simulink model "network_model"  (R2022b)
settings: Solver=ode23t  StartTime=0.0  StopTime=50  FixedStep=1e-3  RelTol=1e-3
values from neighbouring files (symbols this model uses):
  a = 0.9    [network_control.m]
  B = 8    [network_control.m]
  C = 6    [network_control.m]
  k1 = 0.4    [network_control.m]
  k2 = 0.8    [network_control.m]
  k3 = 0.1    [network_control.m]
  q_i_1 = [-2 2 0]'    [network_control.m]
  q_i_2 = [-4 4 0]'    [network_control.m]
  taup = 0    [network_control.m]
  Ts = 0.01    [network_control.m]
libraries: robotmobilelib x2
settings Model: Creator=danie  LastModifiedBy=gaetano
settings OptimizationCC: ReuseModelBlockBuffer=on

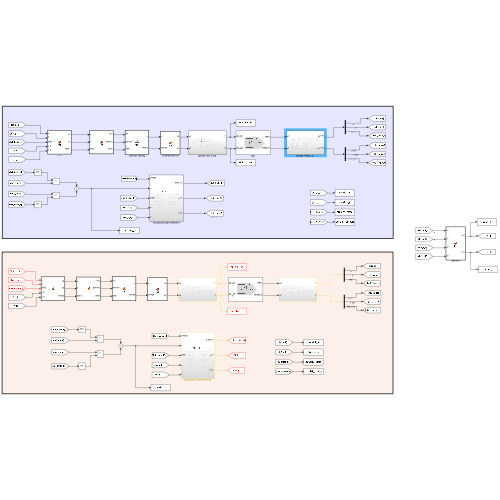
[thumbnail: Simulink's stored preview of the top-level diagram]
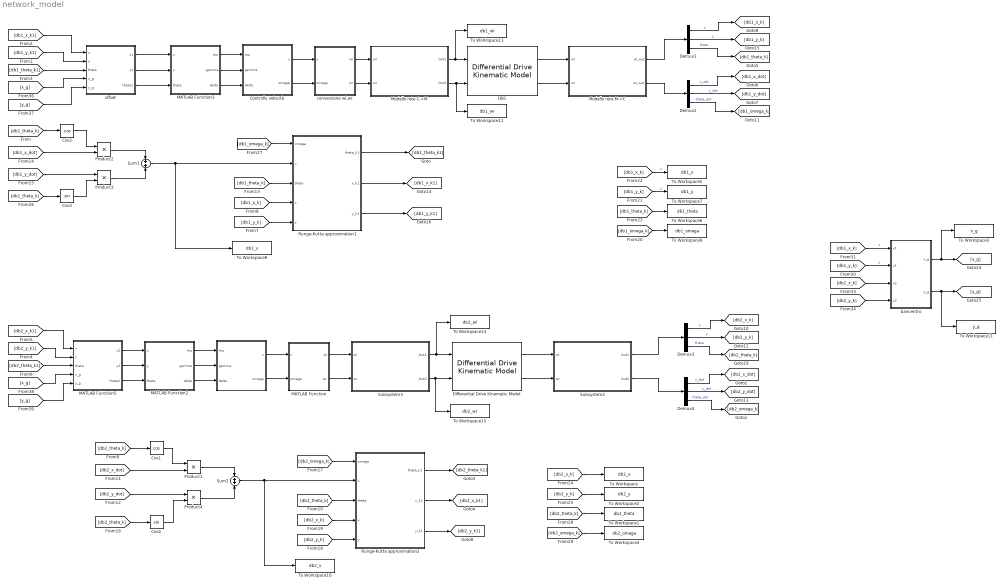
== system network_model ==
  " " : MATLAB Function  TreatAsAtomicUnit=on
  " Controllo velocità" : MATLAB Function  TreatAsAtomicUnit=on
  Cos1 : Trigonometry  Operator=cos
  Cos2 : Trigonometry  Operator=cos
  Cos3 : Trigonometry
  Cos4 : Trigonometry
  DB1 : robotmobilelib/Differential Drive Kinematic Model  VehicleInputs=Wheel Speeds  WheelRadius=0.0318  WheelSpeedRange=[-inf inf]  TrackWidth=0.1232  InitialState=q_i_1  SimulateUsing=Code generation
  Demux{1..4} (4 alike) : Demux  Outputs=3
  Differential Drive Kinematic Model : robotmobilelib/Differential Drive Kinematic Model  VehicleInputs=Wheel Speeds  WheelRadius=0.0318  WheelSpeedRange=[-inf inf]  TrackWidth=0.1232  InitialState=q_i_2  SimulateUsing=Interpreted execution
  MATLAB Function : MATLAB Function  TreatAsAtomicUnit=on
  MATLAB Function2 : MATLAB Function  TreatAsAtomicUnit=on
  MATLAB Function3 : MATLAB Function  TreatAsAtomicUnit=on
  MATLAB Function5 : MATLAB Function  TreatAsAtomicUnit=on
  Modello rete C->M : Subsystem
  Modello rete M->C : Subsystem
  Product{1..4} (4 alike) : Product
  Runge-Kutta approximation1 : Subsystem
  Runge-Kutta approximation2 : Subsystem
  Subsystem2 : Subsystem
  Subsystem3 : Subsystem
  Sum1 : Sum  Inputs=+|+
  Sum2 : Sum  Inputs=+|+
  To Workspace : ToWorkspace  VariableName=db2_x  SaveFormat=Timeseries  SampleTime=-1
  To Workspace1 : ToWorkspace  VariableName=db2_theta  SaveFormat=Timeseries  SampleTime=-1
  To Workspace10 : ToWorkspace  VariableName=db2_v  SaveFormat=Timeseries  SampleTime=-1
  To Workspace11 : ToWorkspace  VariableName=y_g  SaveFormat=Timeseries  SampleTime=-1
  To Workspace12 : ToWorkspace  VariableName=db1_wr  SaveFormat=Timeseries  SampleTime=-1
  To Workspace13 : ToWorkspace  VariableName=db1_wl  SaveFormat=Timeseries  SampleTime=-1
  To Workspace14 : ToWorkspace  VariableName=db2_wl  SaveFormat=Timeseries  SampleTime=-1
  To Workspace15 : ToWorkspace  VariableName=db2_wr  SaveFormat=Timeseries  SampleTime=-1
  To Workspace2 : ToWorkspace  VariableName=db2_y  SaveFormat=Timeseries  SampleTime=-1
  To Workspace3 : ToWorkspace  VariableName=x_g  SaveFormat=Timeseries  SampleTime=-1
  To Workspace4 : ToWorkspace  VariableName=db2_omega  SaveFormat=Timeseries  SampleTime=-1
  To Workspace5 : ToWorkspace  VariableName=db1_x  SaveFormat=Timeseries  SampleTime=-1
  To Workspace6 : ToWorkspace  VariableName=db1_theta  SaveFormat=Timeseries  SampleTime=-1
  To Workspace7 : ToWorkspace  VariableName=db1_y  SaveFormat=Timeseries  SampleTime=-1
  To Workspace8 : ToWorkspace  VariableName=db1_v  SaveFormat=Timeseries  SampleTime=-1
  To Workspace9 : ToWorkspace  VariableName=db1_omega  SaveFormat=Timeseries  SampleTime=-1
  baricentro : MATLAB Function  TreatAsAtomicUnit=on
  conversione wl,wr : MATLAB Function  TreatAsAtomicUnit=on
  offset : MATLAB Function  TreatAsAtomicUnit=on
  wires:
  MATLAB Function3/3(delta) -> " Controllo velocità"/3(delta)
  [db1_theta_k] -> To Workspace6/1
  [db2_y_k] -> Runge-Kutta approximation2/5(y)
  Runge-Kutta approximation2/2(x_k1) -> [db2_x_k1]
  " "/2(omega) -> MATLAB Function/2(omega)
  [db1_y_k] -> Runge-Kutta approximation1/5(y)
  Runge-Kutta approximation2/3(y_k1) -> [db2_y_k1]
  Demux2/1 -> [db1_x_dot]  "x_dot"
  [db1_omega_k] -> Runge-Kutta approximation1/1(omega)
  [db1_theta_k] -> Cos2/1
  Demux1/3 -> [db1_theta_k]  "theta"
  [db1_theta_k] -> Cos3/1
  Product1/1 -> Sum2/1
  Cos1/1 -> Product1/1
  Cos3/1 -> Product3/2
  [db2_theta_k] -> Runge-Kutta approximation2/3(theta)
  Product4/1 -> Sum2/2
  Cos4/1 -> Product4/2
  " Controllo velocità"/1(v) -> conversione wl,wr/1(v)
  Demux1/2 -> [db1_y_k]  "y"
  Demux2/3 -> [db1_omega_k]  "theta_dot"
  Cos2/1 -> Product2/1
  offset/2(y1) -> MATLAB Function3/2(y)
  Demux1/1 -> [db1_x_k]  "x"
  [db1_x_dot] -> Product2/2
  [db1_x_k] -> Runge-Kutta approximation1/4(x)
  Runge-Kutta approximation1/1(theta_k1) -> [db1_theta_k1]
  MATLAB Function3/1(rho) -> " Controllo velocità"/1(rho)
  MATLAB Function2/2(gamma) -> " "/2(gamma)
  " "/1(v) -> MATLAB Function/1(v)
  Demux4/1 -> [db2_x_dot]  "x_dot"
  Product3/1 -> Sum1/2
  [db2_y_k] -> To Workspace2/1
  Sum2/1 -> To Workspace10/1, Runge-Kutta approximation2/2(v)
  [db1_theta_k] -> Runge-Kutta approximation1/3(theta)
  Product2/1 -> Sum1/1
  Demux3/1 -> [db2_x_k]  "x"
  [db2_theta_k] -> Cos4/1
  offset/3(theta1) -> MATLAB Function3/3(theta)
  [db1_y_k] -> baricentro/2(y1)  "y"
  [db1_x_k] -> baricentro/1(x1)  "x"
  MATLAB Function2/1(rho) -> " "/1(rho)
  Sum1/1 -> To Workspace8/1, Runge-Kutta approximation1/2(v)
  [db2_x_k] -> baricentro/3(x2)
  Demux4/3 -> [db2_omega_k]  "theta_dot"
  [db2_omega_k] -> To Workspace4/1
  " Controllo velocità"/2(omega) -> conversione wl,wr/2(omega)
  [db1_y_k1] -> offset/2(y)
  [db2_omega_k] -> Runge-Kutta approximation2/1(omega)
  Demux3/3 -> [db2_theta_k]  "theta"
  [db2_theta_k1] -> MATLAB Function5/3(theta)
  [db2_y_k1] -> MATLAB Function5/2(y)
  MATLAB Function5/1(x2) -> MATLAB Function2/1(x)
  MATLAB Function3/2(gamma) -> " Controllo velocità"/2(gamma)
  [db1_x_k] -> To Workspace5/1  "x"
  [y_g] -> offset/5(y_g)
  [db2_x_k] -> To Workspace/1
  [db1_x_k1] -> offset/1(x)
  Runge-Kutta approximation1/3(y_k1) -> [db1_y_k1]
  [x_g] -> offset/4(x_g)
  [db2_x_k1] -> MATLAB Function5/1(x)
  [db1_y_dot] -> Product3/1
  MATLAB Function5/2(y2) -> MATLAB Function2/2(y)
  [y_g] -> MATLAB Function5/5(y_g)
  [db2_theta_k] -> To Workspace1/1
  [db1_y_k] -> To Workspace7/1  "y"
  [x_g] -> MATLAB Function5/4(x_g)
  [db1_theta_k1] -> offset/3(theta)
  offset/1(x1) -> MATLAB Function3/1(x)
  baricentro/2(y_g) -> [y_g], To Workspace11/1
  [db2_x_k] -> Runge-Kutta approximation2/4(x)
  Demux3/2 -> [db2_y_k]  "y"
  [db2_y_dot] -> Product4/1
  [db2_theta_k] -> Cos1/1
  Demux4/2 -> [db2_y_dot]  "y_dot"
  [db1_omega_k] -> To Workspace9/1
  Runge-Kutta approximation1/2(x_k1) -> [db1_x_k1]
  Demux2/2 -> [db1_y_dot]  "y_dot"
  [db2_x_dot] -> Product1/2
  MATLAB Function2/3(delta) -> " "/3(delta)
  Runge-Kutta approximation2/1(theta_k1) -> [db2_theta_k1]
  baricentro/1(x_g) -> [x_g], To Workspace3/1
  MATLAB Function5/3(theta2) -> MATLAB Function2/3(theta)
  [db2_y_k] -> baricentro/4(y2)
  conversione wl,wr/1(wl) -> Modello rete C->M/1(wl)
  conversione wl,wr/2(wr) -> Modello rete C->M/2(wr)
  Modello rete C->M/1(Out1) -> To Workspace13/1, DB1/1
  Modello rete C->M/2(Out2) -> To Workspace12/1, DB1/2
  Modello rete M->C/1(wl_out) -> Demux1/1
  Modello rete M->C/2(wr_out) -> Demux2/1
  DB1/1 -> Modello rete M->C/1(wl)
  DB1/2 -> Modello rete M->C/2(wr)
  Subsystem2/1(Out1) -> Demux3/1
  Subsystem2/2(Out2) -> Demux4/1
  Differential Drive Kinematic Model/2 -> Subsystem2/2(wr)
  Differential Drive Kinematic Model/1 -> Subsystem2/1(wl)
  MATLAB Function/1(wl) -> Subsystem3/1(wl)
  MATLAB Function/2(wr) -> Subsystem3/2(wr)
  Subsystem3/2(Out2) -> To Workspace15/1, Differential Drive Kinematic Model/2
  Subsystem3/1(Out1) -> To Workspace14/1, Differential Drive Kinematic Model/1

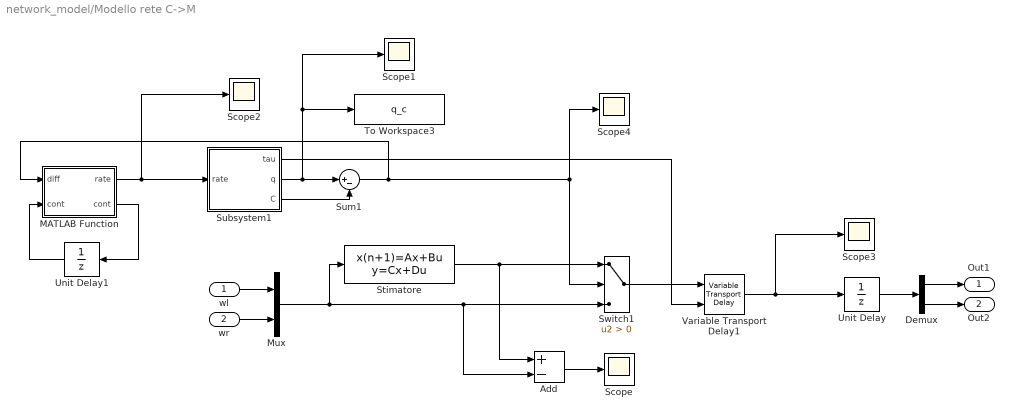
== system network_model/Modello rete C->M ==
  wl : Inport
  wr : Inport  Port=2
  Add : Sum  Inputs=+-
  Demux : Demux  Outputs=2
  MATLAB Function : MATLAB Function  TreatAsAtomicUnit=on
  Mux : Mux  Inputs=2
  Scope{,1..4} (5 alike) : Scope
  Stimatore : DiscreteStateSpace  A=(1-a)*eye(2)  B=a*eye(2)  C=eye(2)  D=zeros(2,2)  SampleTime=-1
  Subsystem1 : Subsystem
  Sum1 : Sum  Inputs=|+-
  Switch1 : Switch  Criteria=u2 > Threshold  SaturateOnIntegerOverflow=off  InputSameDT=off
  To Workspace3 : ToWorkspace  VariableName=q_c  SaveFormat=Timeseries  SampleTime=-1
  Unit Delay : UnitDelay  SampleTime=0.01  HasFrameUpgradeWarning=on
  Unit Delay1 : UnitDelay  SampleTime=-1  HasFrameUpgradeWarning=on
  Variable Transport Delay1 : VariableTransportDelay  MaximumDelay=10  MaximumPoints=2048  ZeroDelay=on
  Out1 : Outport
  Out2 : Outport  Port=2
  wires:
  Switch1/1 -> Variable Transport Delay1/1
  Subsystem1/3(C) -> Sum1/2
  Subsystem1/1(tau) -> Variable Transport Delay1/2
  Subsystem1/2(q) -> To Workspace3/1, Scope1/1, Sum1/1
  Sum1/1 -> MATLAB Function/1(diff), Scope4/1, Switch1/2
  wl/1 -> Mux/1
  wr/1 -> Mux/2
  Mux/1 -> Stimatore/1, Add/2, Switch1/3
  Variable Transport Delay1/1 -> Scope3/1, Unit Delay/1
  Demux/1 -> Out1/1
  Demux/2 -> Out2/1
  Unit Delay/1 -> Demux/1
  Stimatore/1 -> Switch1/1, Add/1
  Add/1 -> Scope/1
  MATLAB Function/1(rate) -> Scope2/1, Subsystem1/1(rate)
  MATLAB Function/2(cont) -> Unit Delay1/1
  Unit Delay1/1 -> MATLAB Function/2("cont ")

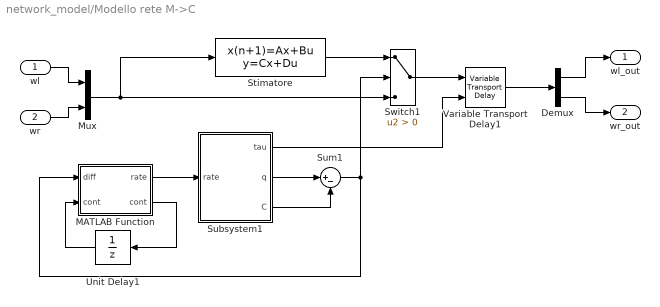
== system network_model/Modello rete M->C ==
  wl : Inport
  wr : Inport  Port=2
  Demux : Demux  Outputs=2
  MATLAB Function : MATLAB Function  TreatAsAtomicUnit=on
  Mux : Mux  Inputs=2
  Stimatore : DiscreteStateSpace  A=(1-a)*eye(6)  B=a*eye(6)  C=eye(6)  D=zeros(6,6)  SampleTime=-1
  Subsystem1 : Subsystem
  Sum1 : Sum  Inputs=|+-
  Switch1 : Switch  Criteria=u2 > Threshold  SaturateOnIntegerOverflow=off  InputSameDT=off
  Unit Delay1 : UnitDelay  SampleTime=-1  HasFrameUpgradeWarning=on
  Variable Transport Delay1 : VariableTransportDelay  MaximumDelay=10  MaximumPoints=2048  ZeroDelay=on
  wl_out : Outport
  wr_out : Outport  Port=2
  wires:
  Demux/2 -> wr_out/1
  Demux/1 -> wl_out/1
  Mux/1 -> Stimatore/1, Switch1/3
  wr/1 -> Mux/2
  wl/1 -> Mux/1
  Subsystem1/2(q) -> Sum1/1
  Subsystem1/1(tau) -> Variable Transport Delay1/2
  Subsystem1/3(C) -> Sum1/2
  Switch1/1 -> Variable Transport Delay1/1
  Variable Transport Delay1/1 -> Demux/1
  Stimatore/1 -> Switch1/1
  MATLAB Function/1(rate) -> Subsystem1/1(rate)
  Sum1/1 -> MATLAB Function/1(diff), Switch1/2
  MATLAB Function/2(cont) -> Unit Delay1/1
  Unit Delay1/1 -> MATLAB Function/2("cont ")

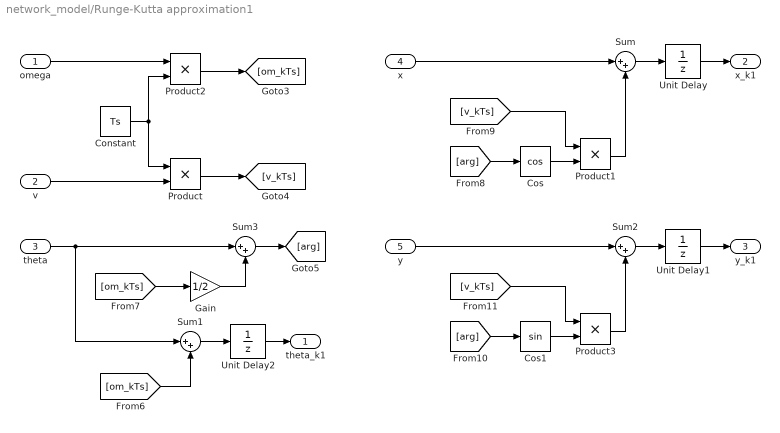
== system network_model/Runge-Kutta approximation1 ==
  omega : Inport
  v : Inport  Port=2
  theta : Inport  Port=3
  x : Inport  Port=4
  y : Inport  Port=5
  Constant : Constant  Value=Ts
  Cos : Trigonometry  Operator=cos
  Cos1 : Trigonometry
  Gain : Gain  Gain=1/2
  Product{,1..3} (4 alike) : Product
  Sum{,1..3} (4 alike) : Sum  Inputs=|++
  Unit Delay : UnitDelay  InitialCondition=q_i_1(1)  SampleTime=Ts  HasFrameUpgradeWarning=on
  Unit Delay1 : UnitDelay  InitialCondition=q_i_1(2)  SampleTime=Ts  HasFrameUpgradeWarning=on
  Unit Delay2 : UnitDelay  InitialCondition=q_i_1(3)  SampleTime=Ts  HasFrameUpgradeWarning=on
  theta_k1 : Outport
  x_k1 : Outport  Port=2
  y_k1 : Outport  Port=3
  wires:
  Sum3/1 -> [arg]
  theta/1 -> Sum1/1, Sum3/1
  [v_kTs] -> Product3/1
  omega/1 -> Product2/1
  [om_kTs] -> Sum1/2
  [arg] -> Cos1/1
  [arg] -> Cos/1
  x/1 -> Sum/1
  Product/1 -> [v_kTs]
  y/1 -> Sum2/1
  [om_kTs] -> Gain/1
  v/1 -> Product/2
  [v_kTs] -> Product1/1
  Cos/1 -> Product1/2
  Constant/1 -> Product2/2, Product/1
  Product2/1 -> [om_kTs]
  Product1/1 -> Sum/2
  Product3/1 -> Sum2/2
  Gain/1 -> Sum3/2
  Cos1/1 -> Product3/2
  Sum1/1 -> Unit Delay2/1
  Sum2/1 -> Unit Delay1/1
  Sum/1 -> Unit Delay/1
  Unit Delay2/1 -> theta_k1/1
  Unit Delay/1 -> x_k1/1
  Unit Delay1/1 -> y_k1/1

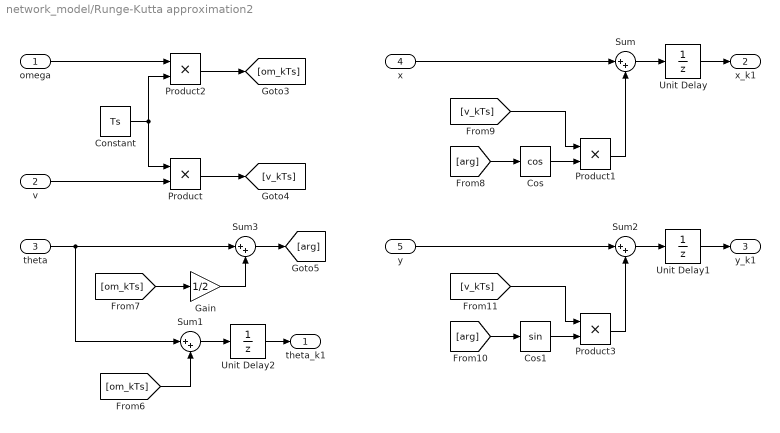
== system network_model/Runge-Kutta approximation2 ==
  omega : Inport
  v : Inport  Port=2
  theta : Inport  Port=3
  x : Inport  Port=4
  y : Inport  Port=5
  Constant : Constant  Value=Ts
  Cos : Trigonometry  Operator=cos
  Cos1 : Trigonometry
  Gain : Gain  Gain=1/2
  Product{,1..3} (4 alike) : Product
  Sum{,1..3} (4 alike) : Sum  Inputs=|++
  Unit Delay : UnitDelay  InitialCondition=q_i_2(1)  SampleTime=Ts  HasFrameUpgradeWarning=on
  Unit Delay1 : UnitDelay  InitialCondition=q_i_2(2)  SampleTime=Ts  HasFrameUpgradeWarning=on
  Unit Delay2 : UnitDelay  InitialCondition=q_i_2(3)  SampleTime=Ts  HasFrameUpgradeWarning=on
  theta_k1 : Outport
  x_k1 : Outport  Port=2
  y_k1 : Outport  Port=3
  wires:
  Sum3/1 -> [arg]
  theta/1 -> Sum1/1, Sum3/1
  [v_kTs] -> Product3/1
  omega/1 -> Product2/1
  [om_kTs] -> Sum1/2
  [arg] -> Cos1/1
  [arg] -> Cos/1
  x/1 -> Sum/1
  Product/1 -> [v_kTs]
  y/1 -> Sum2/1
  [om_kTs] -> Gain/1
  v/1 -> Product/2
  [v_kTs] -> Product1/1
  Cos/1 -> Product1/2
  Constant/1 -> Product2/2, Product/1
  Product2/1 -> [om_kTs]
  Product1/1 -> Sum/2
  Product3/1 -> Sum2/2
  Gain/1 -> Sum3/2
  Cos1/1 -> Product3/2
  Sum1/1 -> Unit Delay2/1
  Sum2/1 -> Unit Delay1/1
  Sum/1 -> Unit Delay/1
  Unit Delay2/1 -> theta_k1/1
  Unit Delay/1 -> x_k1/1
  Unit Delay1/1 -> y_k1/1

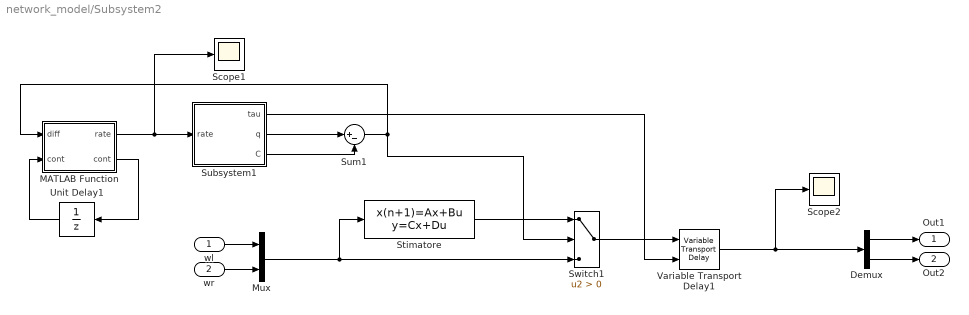
== system network_model/Subsystem2 ==
  wl : Inport
  wr : Inport  Port=2
  Demux : Demux  Outputs=2
  MATLAB Function : MATLAB Function  TreatAsAtomicUnit=on
  Mux : Mux  Inputs=2
  Scope1 : Scope
  Scope2 : Scope
  Stimatore : DiscreteStateSpace  A=(1-a)*eye(6)  B=a*eye(6)  C=eye(6)  D=zeros(6,6)  SampleTime=-1
  Subsystem1 : Subsystem
  Sum1 : Sum  Inputs=|+-
  Switch1 : Switch  Criteria=u2 > Threshold  SaturateOnIntegerOverflow=off  InputSameDT=off
  Unit Delay1 : UnitDelay  SampleTime=-1  HasFrameUpgradeWarning=on
  Variable Transport Delay1 : VariableTransportDelay  MaximumDelay=10  MaximumPoints=2048  ZeroDelay=on
  Out1 : Outport
  Out2 : Outport  Port=2
  wires:
  Switch1/1 -> Variable Transport Delay1/1
  Subsystem1/1(tau) -> Variable Transport Delay1/2
  Subsystem1/2(q) -> Sum1/1
  wl/1 -> Mux/1
  wr/1 -> Mux/2
  Mux/1 -> Stimatore/1, Switch1/3
  Demux/1 -> Out1/1
  Demux/2 -> Out2/1
  Variable Transport Delay1/1 -> Scope2/1, Demux/1
  Stimatore/1 -> Switch1/1
  Subsystem1/3(C) -> Sum1/2
  MATLAB Function/1(rate) -> Subsystem1/1(rate), Scope1/1
  Sum1/1 -> MATLAB Function/1(diff), Switch1/2
  MATLAB Function/2(cont) -> Unit Delay1/1
  Unit Delay1/1 -> MATLAB Function/2("cont ")

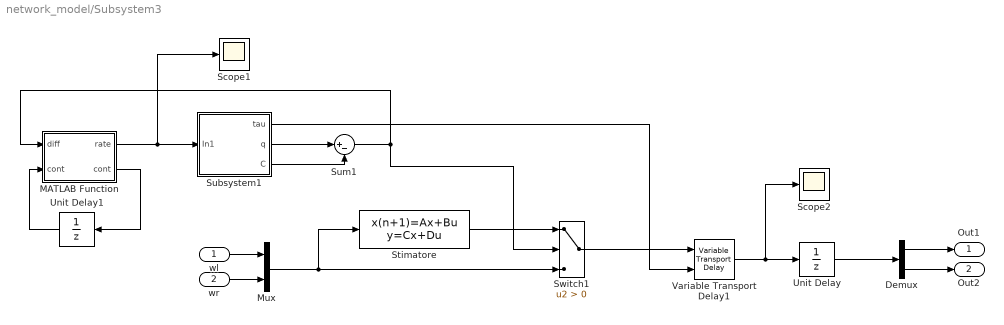
== system network_model/Subsystem3 ==
  wl : Inport
  wr : Inport  Port=2
  Demux : Demux  Outputs=2
  MATLAB Function : MATLAB Function  TreatAsAtomicUnit=on
  Mux : Mux  Inputs=2
  Scope1 : Scope
  Scope2 : Scope
  Stimatore : DiscreteStateSpace  A=(1-a)*eye(2)  B=a*eye(2)  C=eye(2)  D=zeros(2,2)  SampleTime=-1
  Subsystem1 : Subsystem
  Sum1 : Sum  Inputs=|+-
  Switch1 : Switch  Criteria=u2 > Threshold  SaturateOnIntegerOverflow=off  InputSameDT=off
  Unit Delay : UnitDelay  SampleTime=0.01  HasFrameUpgradeWarning=on
  Unit Delay1 : UnitDelay  SampleTime=-1  HasFrameUpgradeWarning=on
  Variable Transport Delay1 : VariableTransportDelay  MaximumDelay=10  MaximumPoints=2048  ZeroDelay=on
  Out1 : Outport
  Out2 : Outport  Port=2
  wires:
  Demux/2 -> Out2/1
  Demux/1 -> Out1/1
  wr/1 -> Mux/2
  wl/1 -> Mux/1
  Subsystem1/2(q) -> Sum1/1
  Subsystem1/1(tau) -> Variable Transport Delay1/2
  Subsystem1/3(C) -> Sum1/2
  Switch1/1 -> Variable Transport Delay1/1
  Mux/1 -> Stimatore/1, Switch1/3
  Variable Transport Delay1/1 -> Scope2/1, Unit Delay/1
  Unit Delay/1 -> Demux/1
  Stimatore/1 -> Switch1/1
  MATLAB Function/1(rate) -> Subsystem1/1(In1), Scope1/1
  Sum1/1 -> MATLAB Function/1(diff), Switch1/2
  MATLAB Function/2(cont) -> Unit Delay1/1
  Unit Delay1/1 -> MATLAB Function/2("cont ")

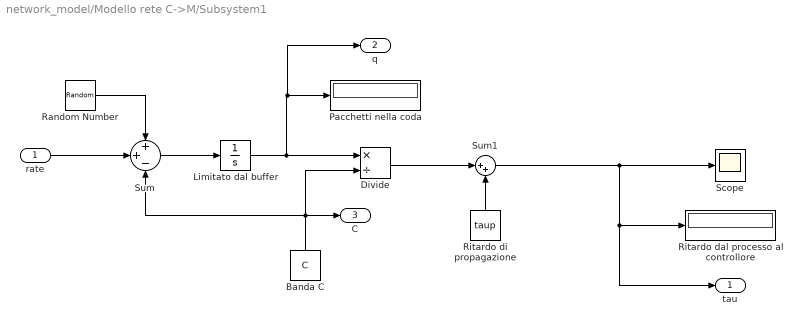
== system network_model/Modello rete C->M/Subsystem1 ==
  rate : Inport
  Banda C : Constant  Value=C
  Divide : Product  Inputs=*/
  Limitato dal buffer : Integrator  LimitOutput=on  UpperSaturationLimit=B  LowerSaturationLimit=0
  Pacchetti nella coda : Display
  Random Number : RandomNumber  Mean=C/2  Variance=C/2  SampleTime=0.01
  Ritardo dal processo al controllore : Display
  Ritardo di propagazione : Constant  Value=taup
  Scope : Scope
  Sum : Sum  Inputs=++-
  Sum1 : Sum  Inputs=|++
  tau : Outport
  q : Outport  Port=2
  C : Outport  Port=3
  wires:
  Sum/1 -> Limitato dal buffer/1
  Limitato dal buffer/1 -> Divide/1, Pacchetti nella coda/1, q/1
  Sum1/1 -> Scope/1, Ritardo dal processo al controllore/1, tau/1
  Ritardo di propagazione/1 -> Sum1/2
  Divide/1 -> Sum1/1
  Banda C/1 -> Sum/3, Divide/2, C/1
  rate/1 -> Sum/2
  Random Number/1 -> Sum/1

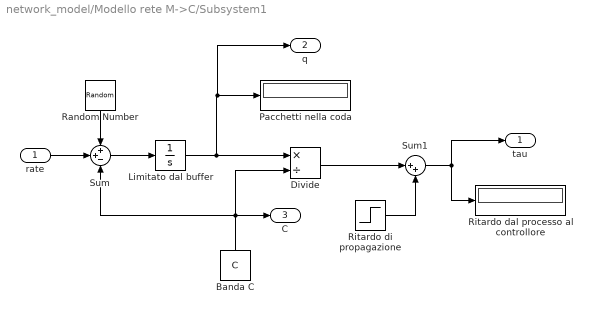
== system network_model/Modello rete M->C/Subsystem1 ==
  rate : Inport
  Banda C : Constant  Value=C
  Divide : Product  Inputs=*/
  Limitato dal buffer : Integrator  LimitOutput=on  UpperSaturationLimit=B  LowerSaturationLimit=0
  Pacchetti nella coda : Display
  Random Number : RandomNumber  Mean=C/2  Variance=C/2  SampleTime=0.01
  Ritardo dal processo al controllore : Display
  Ritardo di propagazione : Step  Time=4*1e-1  After=taup  SampleTime=0
  Sum : Sum  Inputs=++-
  Sum1 : Sum  Inputs=|++
  tau : Outport
  q : Outport  Port=2
  C : Outport  Port=3
  wires:
  Banda C/1 -> Sum/3, Divide/2, C/1
  Divide/1 -> Sum1/1
  Ritardo di propagazione/1 -> Sum1/2
  Sum1/1 -> tau/1, Ritardo dal processo al controllore/1
  Limitato dal buffer/1 -> q/1, Pacchetti nella coda/1, Divide/1
  Sum/1 -> Limitato dal buffer/1
  rate/1 -> Sum/2
  Random Number/1 -> Sum/1

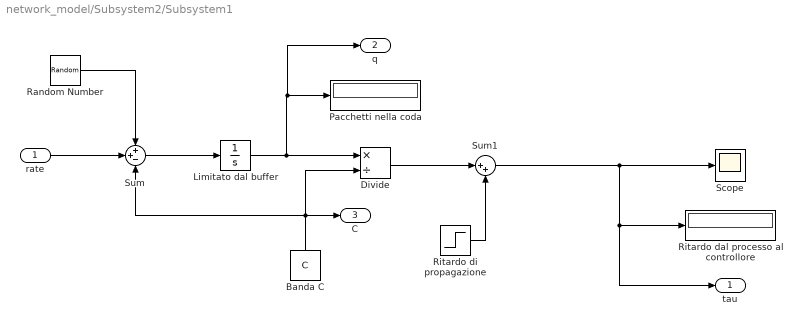
== system network_model/Subsystem2/Subsystem1 ==
  rate : Inport
  Banda C : Constant  Value=C
  Divide : Product  Inputs=*/
  Limitato dal buffer : Integrator  LimitOutput=on  UpperSaturationLimit=B  LowerSaturationLimit=0
  Pacchetti nella coda : Display
  Random Number : RandomNumber  Mean=C/2  Variance=C/2  SampleTime=0.01
  Ritardo dal processo al controllore : Display
  Ritardo di propagazione : Step  Time=4*1e-1  After=taup  SampleTime=0
  Scope : Scope
  Sum : Sum  Inputs=++-
  Sum1 : Sum  Inputs=|++
  tau : Outport
  q : Outport  Port=2
  C : Outport  Port=3
  wires:
  Sum/1 -> Limitato dal buffer/1
  Limitato dal buffer/1 -> Divide/1, Pacchetti nella coda/1, q/1
  Sum1/1 -> Scope/1, Ritardo dal processo al controllore/1, tau/1
  Ritardo di propagazione/1 -> Sum1/2
  Divide/1 -> Sum1/1
  Banda C/1 -> Sum/3, Divide/2, C/1
  rate/1 -> Sum/2
  Random Number/1 -> Sum/1

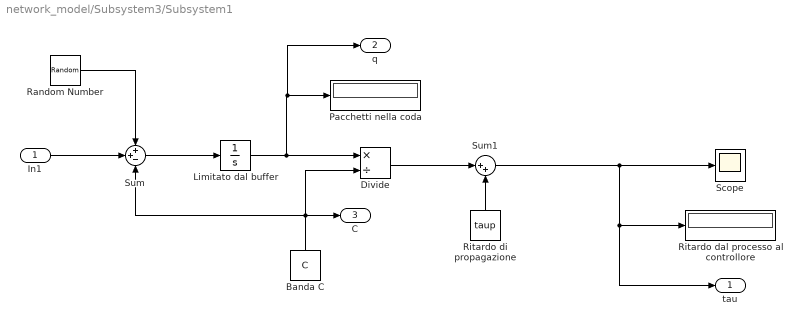
== system network_model/Subsystem3/Subsystem1 ==
  In1 : Inport
  Banda C : Constant  Value=C
  Divide : Product  Inputs=*/
  Limitato dal buffer : Integrator  LimitOutput=on  UpperSaturationLimit=B  LowerSaturationLimit=0
  Pacchetti nella coda : Display
  Random Number : RandomNumber  Mean=C/2  Variance=C/2  SampleTime=0.01
  Ritardo dal processo al controllore : Display
  Ritardo di propagazione : Constant  Value=taup
  Scope : Scope
  Sum : Sum  Inputs=++-
  Sum1 : Sum  Inputs=|++
  tau : Outport
  q : Outport  Port=2
  C : Outport  Port=3
  wires:
  Banda C/1 -> Sum/3, C/1, Divide/2
  Divide/1 -> Sum1/1
  Ritardo di propagazione/1 -> Sum1/2
  Sum1/1 -> tau/1, Ritardo dal processo al controllore/1, Scope/1
  Limitato dal buffer/1 -> q/1, Pacchetti nella coda/1, Divide/1
  Sum/1 -> Limitato dal buffer/1
  In1/1 -> Sum/2
  Random Number/1 -> Sum/1

== matlab function network_model/MATLAB Function5 ==
  data: x input; x2 output; y2 output; y input; theta input; theta2 output; x_g input; y_g input
function [x2,y2,theta2] = fcn(x,y,theta,x_g,y_g)

offx = (x-x_g);
offy = (y-y_g) - 0.7;

x2 = x + offx;
y2 = y + offy;
theta2 = theta;

== matlab function network_model/Modello rete C->M/MATLAB Function ==
  data: diff input; rate output; cont input; cont output
function [rate, cont] = fcn(diff, cont)

rate_min=3;
rate_max=8;

if (diff>0)
    cont=cont+1;
    if(cont==10)
        rate=rate_min;
        cont=0;
    else rate=rate_max;
    end

elseif(diff<=0)
    cont=cont+1;
    if(cont==10)
        rate=rate_max;
        cont=0;
    else rate=rate_min;
    end
else rate=rate_max;
end

end

== matlab function network_model/Modello rete M->C/MATLAB Function ==
  data: diff input; rate output; cont input; cont output
function [rate, cont] = fcn(diff, cont)

rate_min=3;
rate_max=8;

if (diff>0)
    cont=cont+1;
    if(cont==10)
        rate=rate_min;
        cont=0;
    else rate=rate_max;
    end

elseif(diff<=0)
    cont=cont+1;
    if(cont==10)
        rate=rate_max;
        cont=0;
    else rate=rate_min;
    end
else rate=rate_max;
end

end

== matlab function network_model/ Controllo velocità ==
  data: rho input; v output; omega output; gamma input; delta input; k1 parameter; k2 parameter; k3 parameter
function [v,omega] = fcn(rho,gamma,delta, k1, k2, k3)

v = k1 * rho * cos(gamma);
omega = k2 * gamma + k1*sin(gamma)*cos(gamma)*(1+k3*delta/gamma);

== matlab function network_model/Subsystem3/MATLAB Function ==
  data: diff input; rate output; cont input; cont output
function [rate, cont] = fcn(diff, cont)

rate_min=3;
rate_max=8;

if (diff>0)
    cont=cont+1;
    if(cont==10)
        rate=rate_min;
        cont=0;
    else rate=rate_max;
    end

elseif(diff<=0)
    cont=cont+1;
    if(cont==10)
        rate=rate_max;
        cont=0;
    else rate=rate_min;
    end
else rate=rate_max;
end

end

== matlab function network_model/Subsystem2/MATLAB Function ==
  data: diff input; rate output; cont input; cont output
function [rate, cont] = fcn(diff, cont)

rate_min=3;
rate_max=8;

if (diff>0)
    cont=cont+1;
    if(cont==10)
        rate=rate_min;
        cont=0;
    else rate=rate_max;
    end

elseif(diff<=0)
    cont=cont+1;
    if(cont==10)
        rate=rate_max;
        cont=0;
    else rate=rate_min;
    end
else rate=rate_max;
end

end

== matlab function network_model/MATLAB Function ==
  data: wl output; v input; omega input; wr output
function [wl, wr] = fcn(v, omega)

 raggio = 0.0318;
 interasse = 0.1232;

	wr = (2*v + omega*interasse)/(2*raggio);
	wl = (2*v - omega*interasse)/(2*raggio);

end

== matlab function network_model/MATLAB Function2 ==
  data: x input; rho output; gamma output; y input; theta input; delta output
function [rho,gamma,delta] = fcn(x,y,theta)

rho = sqrt(x^2+y^2);

gamma = atan2(y,x) - theta + pi;
% gamma = mod(gamma + pi, 2*pi) - pi;
    while gamma > pi
        gamma = gamma - 2*pi;
    end
    
    while gamma < -pi
        gamma = gamma + 2*pi;
    end

delta = gamma + theta;

== matlab function network_model/  ==
  data: rho input; v output; omega output; gamma input; delta input; k1 parameter; k2 parameter; k3 parameter
function [v,omega] = fcn(rho,gamma,delta, k1, k2, k3)

v = k1 * rho * cos(gamma);
omega = k2 * gamma + k1*sin(gamma)*cos(gamma)*(1+k3*delta/gamma);

== matlab function network_model/conversione wl,wr ==
  data: wl output; v input; omega input; wr output
function [wl, wr] = fcn(v, omega)

 raggio = 0.0318;
 interasse = 0.1232;

	wr = (2*v + omega*interasse)/(2*raggio);
	wl = (2*v - omega*interasse)/(2*raggio);

end

== matlab function network_model/MATLAB Function3 ==
  data: x input; rho output; gamma output; y input; theta input; delta output
function [rho,gamma,delta] = fcn(x,y,theta)

rho = sqrt(x^2+y^2);

gamma = atan2(y,x) - theta + pi;
% gamma = mod(gamma + pi, 2*pi) - pi;
    while gamma > pi
        gamma = gamma - 2*pi;
    end
    
    while gamma < -pi
        gamma = gamma + 2*pi;
    end

delta = gamma + theta;

== matlab function network_model/baricentro ==
  data: x1 input; x_g output; y1 input; x2 input; y2 input; y_g output
function [x_g,y_g] = fcn(x1,y1,x2,y2)

x_g = (x1+x2)/2;
y_g = (y1+y2)/2;

== matlab function network_model/offset ==
  data: x input; x1 output; y1 output; y input; theta input; theta1 output; x_g input; y_g input
function [x1,y1,theta1] = fcn(x,y,theta,x_g,y_g)

offx = (x-x_g);
offy = (y-y_g) + 0.7;

x1 = x + offx;
y1 = y + offy;
theta1 = theta;
